simulink model "BIG_MUFF_PI_inputStage_ssc"  (R2025b)
settings: Solver=VariableStepAuto  StartTime=0  StopTime=5.1  FixedStep=1/96e3  RelTol=1e-3
libraries: fl_lib x17, ee_lib x11, nesl_utility x3
(part 1 of 2)
settings Model: Creator=riccardo
settings SolverCC: AlgebraicLoopSolver=TrustRegion
settings DataIOCC: OutputOption=SpecifiedOutputTimes  OutputTimes=[0;1.04166666666667e-05;2.08333333333333e-05;3.125e-05;4.16666666666667e-05;5.20833333333333e-05;6.25e-05;7.29166666666667e-05;8.33333333333333e-05;9.375e-05;0.000104166666666667;0.000114583333333333;0.000125;0.000135416666666667;0.000145833333333333;0.00015625;0.000166666666666667;0.000177083333333333;0.0001875;0.000197916666666667;0.000208333333333333;0.00021875;0.000229166666666667;0.000239583333333333;0.00025;0.000260416666666667;0.000270833333333333;0.00028125;0.000291666666666667;0.000302083333333333;0.0003125;0.000322916666666667;0.000333333333333333;0.00034375;0.000354166666666667;0.000364583333333333;0.000375;0.000385416666666667;0.000395833333333333;0.00040625;0.000416666666666667;0.000427083333333333;0.0004375;0.000447916666666667;0.000458333333333333;0.00046875;0.000479166666666667;0.000489583333333333;0.0005;0.000510416666666667;0.000520833333333333;0.00053125;0.000541666666666667;0.000552083333333333;0.0005625;0.000572916666666667;0.000583333333333333;0.00059375;0.000604166666666667;0.000614583333333333;0.000625;0.000635416666666667;0.000645833333333333;0.00065625;0.000666666666666667;0.000677083333333333;0.0006875;0.000697916666666667;0.000708333333333333;0.00071875;0.000729166666666667;0.000739583333333333;0.00075;0.000760416666666667;0.000770833333333333;0.00078125;0.000791666666666667;0.000802083333333333;0.0008125;0.000822916666666667;0.000833333333333333;0.00084375;0.000854166666666667;0.000864583333333333;0.000875;0.000885416666666667;0.000895833333333333;0.00090625;0.000916666666666667;0.000927083333333333;0.0009375;0.000947916666666667;0.000958333333333333;0.00096875;0.000979166666666667;0.000989583333333333;0.001;0.00101041666666667;0.00102083333333333;0.00103125;0.00104166666666667;0.00105208333333333;0.0010625;0.00107291666666667;0.00108333333333333;0.00109375;0.00110416666666667;0.00111458333333333;0.001125;0.00113541666666667;0.00114583333333333;0.00115625;0.00116666666666667;0.00117708333333333;0.0011875;0.00119791666666667;0.00120833333333333;0.00121875;0.00122916666666667;0.00123958333333333;0.00125;0.00126041666666667;0.00127083333333333;0.00128125;0.00129166666666667;0.00130208333333333;0.0013125;0.00132291666666667;0.00133333333333333;0.00134375;0.00135416666666667;0.00136458333333333;0.001375;0.00138541666666667;0.00139583333333333;0.00140625;0.00141666666666667;0.00142708333333333;0.0014375;0.00144791666666667;0.00145833333333333;0.00146875;0.00147916666666667;0.00148958333333333;0.0015;0.00151041666666667;0.00152083333333333;0.00153125;0.00154166666666667;0.00155208333333333;0.0015625;0.00157291666666667;0.00158333333333333;0.00159375;0.00160416666666667;0.00161458333333333;0.001625;0.00163541666666667;0.00164583333333333;0.00165625;0.00166666666666667;0.00167708333333333;0.0016875;0.00169791666666667;0.00170833333333333;0.00171875;0.00172916666666667;0.00173958333333333;0.00175;0.00176041666666667;0.00177083333333333;0.00178125;0.00179166666666667;0.00180208333333333;0.0018125;0.00182291666666667;0.00183333333333333;0.00184375;0.00185416666666667;0.00186458333333333;0.001875;0.00188541666666667;0.00189583333333333;0.00190625;0.00191666666666667;0.00192708333333333;0.0019375;0.00194791666666667;0.00195833333333333;0.00196875;0.00197916666666667;0.00198958333333333;0.002;0.00201041666666667;0.00202083333333333;0.00203125;0.00204166666666667;0.00205208333333333;0.0020625;0.00207291666666667;0.00208333333333333;0.00209375;0.00210416666666667;0.00211458333333333;0.002125;0.00213541666666667;0.00214583333333333;0.00215625;0.00216666666666667;0.00217708333333333;0.0021875;0.00219791666666667;0.00220833333333333;0.00221875;0.00222916666666667;0.00223958333333333;0.00225;0.00226041666666667;0.00227083333333333;0.00228125;0.00229166666666667;0.00230208333333333;0.0023125;0.00232291666666667;0.00233333333333333;0.00234375;0.00235416666666667;0.00236458333333333;0.002375;0.00238541666666667;0.00239583333333333;0.00240625;0.00241666666666667;0.00242708333333333;0.0024375;0.00244791666666667 ...(+7252444 chars)]  ReturnWorkspaceOutputsName=tp19cb4a2c_3148_4d73_bbe6_9ae95a49d26c
settings OptimizationCC: ReuseModelBlockBuffer=off
settings DebuggingCC: UnconnectedInputMsg=warning  UnconnectedOutputMsg=warning  UnconnectedLineMsg=warning
settings ModelReferenceCC: EnableRefExpFcnMdlSchedulingChecks=on
settings RTWCC: GPUComputeCapability=3.5

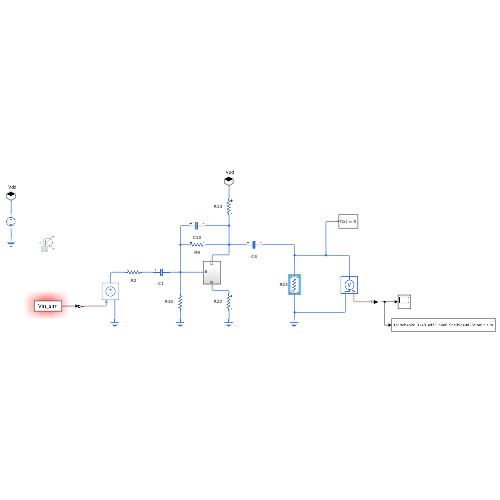
[thumbnail: Simulink's stored preview of the top-level diagram]
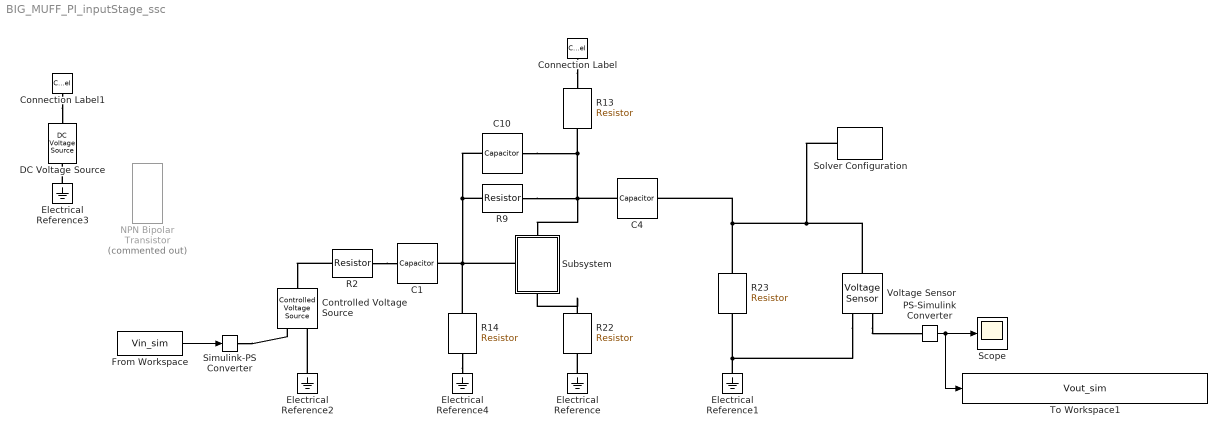
== system BIG_MUFF_PI_inputStage_ssc ==
  C1 : fl_lib/Electrical/Electrical Elements/Capacitor  c=1e-6 F  r=0 Ohm  g=0 1/Ohm  i_specify=off  i_priority=None  i=0 A  i_nominal_specify=off  i_nominal_value=1  i_nominal_unit=A  v_specify=off  v_priority=None  v=0 V  v_nominal_specify=off  v_nominal_value=1  v_nominal_unit=V  vc_specify=off  vc_priority=High  vc=0 V  vc_nominal_specify=off  vc_nominal_value=1  vc_nominal_unit=V
  C10 : fl_lib/Electrical/Electrical Elements/Capacitor  c=470e-12 F  r=0 Ohm  g=0 1/Ohm  i_specify=off  i_priority=None  i=0 A  i_nominal_specify=off  i_nominal_value=1  i_nominal_unit=A  v_specify=off  v_priority=None  v=0 V  v_nominal_specify=off  v_nominal_value=1  v_nominal_unit=V  vc_specify=off  vc_priority=High  vc=0 V  vc_nominal_specify=off  vc_nominal_value=1  vc_nominal_unit=V
  C4 : fl_lib/Electrical/Electrical Elements/Capacitor  c=1e-6 F  r=0 Ohm  g=0 1/Ohm  i_specify=off  i_priority=None  i=0 A  i_nominal_specify=off  i_nominal_value=1  i_nominal_unit=A  v_specify=off  v_priority=None  v=0 V  v_nominal_specify=off  v_nominal_value=1  v_nominal_unit=V  vc_specify=off  vc_priority=High  vc=0 V  vc_nominal_specify=off  vc_nominal_value=1  vc_nominal_unit=V
  Connection Label : ConnectionLabel  Label=Vdd
  Connection Label1 : ConnectionLabel  Label=Vdd
  Controlled Voltage Source : fl_lib/Electrical/Electrical Sources/Controlled Voltage Source
  DC Voltage Source : fl_lib/Electrical/Electrical Sources/DC Voltage Source  v0=9 V
  Electrical Reference{,1..4} (5 alike) : fl_lib/Electrical/Electrical Elements/Electrical Reference
  From Workspace : FromWorkspace  VariableName=Vin_sim
  NPN Bipolar Transistor : ee_lib/Semiconductors & Converters/NPN Bipolar Transistor  Commented=on  parameterization=2  BF=236  IS=33.58e-15 A  VAF=Inf V  hfe=100  hoe=50e-6 1/Ohm  Ic_h=1 mA  Vce_h=5 V  V1=0.55 V  I1=0.5 mA  BR=5.774  Tmeas=28 degC  RC=0 Ohm  RE=0 Ohm  RB=0 Ohm  C_BC=0 pF  C_BE=0 pF  TF=0 us  TR=0 us  prmDatasheet=1  prmEquCoeff=1  hfe_T2=125  XTB=0  V1_T2=0.45 V  I1_T2=0.5 mA  Tmeas2=125 degC  EG=1.11 eV  XTI=3  TdeviceDatasheet=25 degC  TdeviceEquCoeff=25 degC  ec=1  ib_specify=off  ib_priority=None  ib=0 A  ib_nominal_specify=off  ib_nominal_value=1  ib_nominal_unit=A  ic_specify=off  ic_priority=None  ic=0 A  ic_nominal_specify=off  ic_nominal_value=1  ic_nominal_unit=A  vce_specify=off  vce_priority=None  vce=0 V  vce_nominal_specify=off  vce_nominal_value=1  vce_nominal_unit=V  vbe_specify=off  vbe_priority=None  vbe=0 V  vbe_nominal_specify=off  vbe_nominal_value=1  vbe_nominal_unit=V  Qbc_specify=off  Qbc_priority=High  Qbc=0 C  Qbc_nominal_specify=off  Qbc_nominal_value=1  Qbc_nominal_unit=uC  Qbe_specify=off  Qbe_priority=High  Qbe=0 C  Qbe_nominal_specify=off  Qbe_nominal_value=1  Qbe_nominal_unit=uC  thermal_network_parameterization=ee.enum.thermalNetworkTopology.junctionCase  Rth=[0, 10] K/W  Rth_Cauer=[1, 3, 10] K/W  Rth_Foster=[4, 6] K/W  thermal_mass_parameterization=ee.enum.thermalNetwork.timeconstant  thermal_mass=[0, 1] J/K  thermal_mass_Cauer=[.1, .3, 1] J/K  thermal_mass_Foster=[1.5, 3] J/K  thermal_time_constant=[0, 10] s  thermal_time_constant_Cauer=[1, 3, 10] s  thermal_time_constant_Foster=[6, 18] s  thermal_mass_initial_temperatures=[25, 25] degC  thermal_mass_initial_temperatures_Cauer=[25, 25, 25] degC  Tvec_initial_Foster=[25, 25, 25, 25] degC
      settings: InternalSimscapePortConfiguration="{\"Bottom\":[],\"Left\":[{\"id\":\"B\",\"label\":\"\",\"type\":\"foundation.electrical.electrical\"}],\"Right\":[{\"id\":\"C\",\"label\":\"\",\"type\":\"foundation.electrical.electrical\"},{\"id\":\"E\",\"label\":\"\",\"type\":\"foundation.electrical.electrical\"}],\"Top\":[]}"
  PS-Simulink Converter : nesl_utility/PS-Simulink Converter  PhysicalDomain=network_engine_domain  SubClassName=ps_output  LeftPortType=input  RightPortType=output  PseudoPeriodic=off  Frequencies=[]  VectorFormat=1-D array  Unit=inherit  AffineConversion=off
  R13 : ee_lib/Passive/Resistor  R=1e4 Ohm  enable_R_tol=0  R_tol=5  tol_distribution=1  nSigma=4  enable_operating_limits=0  operating_limit_action=2  power_rating=1 W  max_working_voltage=100 V  noise_mode=0  Tdevice=25 degC  sample_time=1e-3 s  repeatability=1  user_seed=0  auto_seed=4112460543  power_derating_T1=70 degC  power_derating_T2=155 degC  operating_temperature_range_vec=[-50, 150] degC  alpha=3.93e-3 1/K  Tmeas=25 degC  thermal_mass=100 J/K  temperature_specify=off  temperature_priority=High  temperature=298.15 K  temperature_nominal_specify=off  temperature_nominal_value=1  temperature_nominal_unit=K
  R14 : ee_lib/Passive/Resistor  R=47e3 Ohm  enable_R_tol=0  R_tol=5  tol_distribution=1  nSigma=4  enable_operating_limits=0  operating_limit_action=2  power_rating=1 W  max_working_voltage=100 V  noise_mode=0  Tdevice=25 degC  sample_time=1e-3 s  repeatability=1  user_seed=0  auto_seed=3499211588  power_derating_T1=70 degC  power_derating_T2=155 degC  operating_temperature_range_vec=[-50, 150] degC  alpha=3.93e-3 1/K  Tmeas=25 degC  thermal_mass=100 J/K  temperature_specify=off  temperature_priority=High  temperature=298.15 K  temperature_nominal_specify=off  temperature_nominal_value=1  temperature_nominal_unit=K
  R2 : ee_lib/Passive/Resistor  R=39e3 Ohm  enable_R_tol=0  R_tol=5  tol_distribution=1  nSigma=4  enable_operating_limits=0  operating_limit_action=2  power_rating=1 W  max_working_voltage=100 V  noise_mode=0  Tdevice=25 degC  sample_time=1e-3 s  repeatability=1  user_seed=0  auto_seed=418932850  power_derating_T1=70 degC  power_derating_T2=155 degC  operating_temperature_range_vec=[-50, 150] degC  alpha=3.93e-3 1/K  Tmeas=25 degC  thermal_mass=100 J/K  temperature_specify=off  temperature_priority=High  temperature=298.15 K  temperature_nominal_specify=off  temperature_nominal_value=1  temperature_nominal_unit=K
  R22 : ee_lib/Passive/Resistor  R=100 Ohm  enable_R_tol=0  R_tol=5  tol_distribution=1  nSigma=4  enable_operating_limits=0  operating_limit_action=2  power_rating=1 W  max_working_voltage=100 V  noise_mode=0  Tdevice=25 degC  sample_time=1e-3 s  repeatability=1  user_seed=0  auto_seed=1196140742  power_derating_T1=70 degC  power_derating_T2=155 degC  operating_temperature_range_vec=[-50, 150] degC  alpha=3.93e-3 1/K  Tmeas=25 degC  thermal_mass=100 J/K  temperature_specify=off  temperature_priority=High  temperature=298.15 K  temperature_nominal_specify=off  temperature_nominal_value=1  temperature_nominal_unit=K
  R23 : ee_lib/Passive/Resistor  R=101e3 Ohm  enable_R_tol=0  R_tol=5  tol_distribution=1  nSigma=4  enable_operating_limits=0  operating_limit_action=2  power_rating=1 W  max_working_voltage=100 V  noise_mode=0  Tdevice=25 degC  sample_time=1e-3 s  repeatability=1  user_seed=0  auto_seed=2348838240  power_derating_T1=70 degC  power_derating_T2=155 degC  operating_temperature_range_vec=[-50, 150] degC  alpha=3.93e-3 1/K  Tmeas=25 degC  thermal_mass=100 J/K  temperature_specify=off  temperature_priority=High  temperature=298.15 K  temperature_nominal_specify=off  temperature_nominal_value=1  temperature_nominal_unit=K
  R9 : ee_lib/Passive/Resistor  R=470e3 Ohm  enable_R_tol=0  R_tol=5  tol_distribution=1  nSigma=4  enable_operating_limits=0  operating_limit_action=2  power_rating=1 W  max_working_voltage=100 V  noise_mode=0  Tdevice=25 degC  sample_time=1e-3 s  repeatability=1  user_seed=0  auto_seed=3890346746  power_derating_T1=70 degC  power_derating_T2=155 degC  operating_temperature_range_vec=[-50, 150] degC  alpha=3.93e-3 1/K  Tmeas=25 degC  thermal_mass=100 J/K  temperature_specify=off  temperature_priority=High  temperature=298.15 K  temperature_nominal_specify=off  temperature_nominal_value=1  temperature_nominal_unit=K
  Scope : Scope
      settings: ActiveDisplayYMinimum=-4.57402  ActiveDisplayYMaximum=9.39625
  Simulink-PS Converter : nesl_utility/Simulink-PS Converter  PhysicalDomain=network_engine_domain  SubClassName=ps_input  LeftPortType=input  RightPortType=output  PseudoPeriodic=off  Frequencies=[]  NoiseDistribution=none  NoiseParameters=[]  Unit=1  AffineConversion=off  FilteringAndDerivatives=provide  SimscapeFilterOrder=1  InputFilterTimeConstant=0.001  UdotUserProvided=0
  Solver Configuration : nesl_utility/Solver Configuration  PhysicalDomain=network_engine_domain  SubClassName=solver  LeftPortType=input  RightPortType=generic  Tones=[]  Harmonics=[]  SimulateNoise=off  Profile=off  UseLocalSampling=off  EnableSwitchedLinearOptims=on  FrequencyDomain=off  UseCCode=off  RelTol=0.001  AbsTol=1e-06  MinStep=1e-09  ToWorkspace=off  RevertToSquareIcSolve=off  NumHomotopyIterations=100  PhasorMode=off  PhasorModeNumHarmonics=1  ConsistencySolver=NEWTON_FTOL  IndexReductionMethod=DerivativeReplacement  DoDC=off  ResidualTolerance=1e-9  ConsistencyTolSource=GLOBAL  ConsistencyAbsTol=0.001  ConsistencyRelTol=0.001  ConsistencyTolFactor=0.001  UseLocalSolver=off  LocalSolverChoice=NE_BACKWARD_EULER_ADVANCER  ResolveIndetEquations=on  FunctionEvalNumThread=1  LocalSolverSampleTime=0.001  DoFixedCost=off  MaxNonlinIter=3  MaxModeIter=2  ComputeImpulses=off  ImpulseIterations=2  LinearAlgebra=auto  LinearAlgebraNumThread=0  EquationFormulation=NE_TIME_EF  DelaysMemoryBudget=1024  AutomaticFiltering=on  FilteringTimeConstant=0.001  PartitionStorageMethod=AS_NEEDED  PartitionMemoryBudget=1024  PartitionMethod=ROBUST  MultibodyUseLocalSolver=off  MultibodyLocalSolverChoice=ODE1  MultibodyLocalSolverSampleTime=0.001
  Subsystem : Subsystem
      settings: PortSchema="{\"entries\":[{\"content\":{\"sides\":[{\"content\":{\"connectorIds\":[\"LConn1\"]},\"type\":\"ConnectorPlacement.EquallySpacedRectSide\",\"uuid\":\"e7d2ad01-b729-4278-a2af-615928332c77\"},{\"content\":{\"connectorIds\":[],\"side\":\"RIGHT\"},\"type\":\"ConnectorPlacement.EquallySpacedRectSide\",\"uuid\":\"6c8f5083-1d74-476b-8fc8-74f7e6a90163\"},{\"content\":{\"connectorIds\":[\"LConn2\"],\"side\":\"TOP\"},\"type\":\"ConnectorPlacement.EquallySpacedRectSide\",\"uuid\":\"cf8d2faf-1e25-415e-bca0-3701d5262d4d\"},{\"content\":{\"connectorIds\":[\"RConn1\"],\"side\":\"BOTTOM\"},\"type\":\"ConnectorPlacement.EquallySpacedRectSide\",\"uuid\":\"80ad8aee-c458-4554-96ef-dc25eb201335\"}]},\"type\":\"ConnectorPlacement.EquallySpacedConnector\",\"uuid\":\"23596b54-1579-47cb-b7ec-00e276fa3e81\"}],\"packageUris\":[\"http://schema.mathworks.com/mf0/Connector/19700101\"],\"version\":\"1.0\"}"
  To Workspace1 : ToWorkspace  VariableName=Vout_sim  SampleTime=-1
  Voltage Sensor : fl_lib/Electrical/Electrical Sensors/Voltage Sensor
  wires:
  PS-Simulink Converter/1 -> To Workspace1/1, Scope/1
  From Workspace/1 -> Simulink-PS Converter/1
  connections:
  Subsystem/LConn1 -- C10/LConn1 -- R9/LConn1 -- R14/LConn1 -- C1/RConn1
  R2/RConn1 -- C1/LConn1
  R22/LConn1 -- Subsystem/RConn1
  Subsystem/LConn2 -- C4/LConn1 -- R9/RConn1 -- C10/RConn1 -- R13/RConn1
  Connection Label/LConn1 -- R13/LConn1
  Electrical Reference/LConn1 -- R22/RConn1
  Electrical Reference1/LConn1 -- Voltage Sensor/RConn2 -- R23/RConn1
  R2/LConn1 -- Controlled Voltage Source/LConn1
  Electrical Reference2/LConn1 -- Controlled Voltage Source/RConn2
  Electrical Reference3/LConn1 -- DC Voltage Source/RConn1
  Connection Label1/LConn1 -- DC Voltage Source/LConn1
  Voltage Sensor/RConn1 -- PS-Simulink Converter/LConn1
  R14/RConn1 -- Electrical Reference4/LConn1
  Solver Configuration/RConn1 -- Voltage Sensor/LConn1 -- R23/LConn1 -- C4/RConn1
  Simulink-PS Converter/RConn1 -- Controlled Voltage Source/RConn1
